simulink model "Scoped_In"  (R2025b)
settings: Solver=VariableStepAuto  StartTime=0.0  StopTime=10.0  RelTol=1e-3
settings Model: Creator=EMK7KOR  LastModifiedBy=EMK7KOR

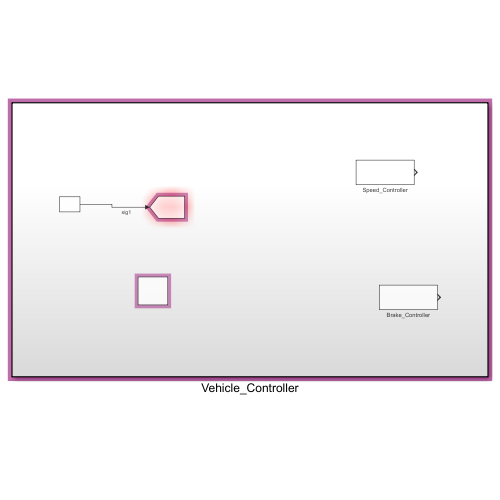
[thumbnail: Simulink's stored preview of the top-level diagram]
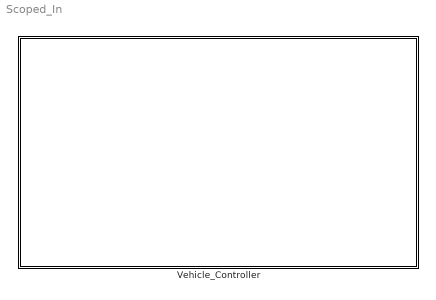
== system Scoped_In ==
  Vehicle_Controller : Subsystem

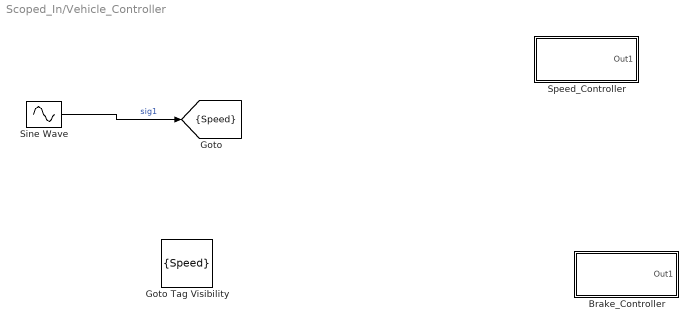
== system Scoped_In/Vehicle_Controller ==
  Brake_Controller : Subsystem
  Goto Tag Visibility : GotoTagVisibility  GotoTag=Speed
  Sine Wave : Sin  SampleTime=0
  Speed_Controller : Subsystem
  tag scope: Speed=scoped
  wires:
  Sine Wave/1 -> [Speed]  "sig1"

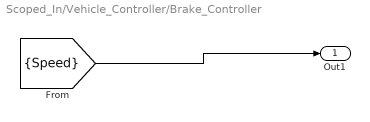
== system Scoped_In/Vehicle_Controller/Brake_Controller ==
  Out1 : Outport
  wires:
  [Speed] -> Out1/1

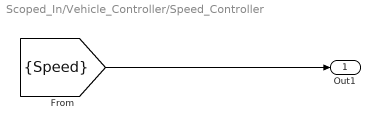
== system Scoped_In/Vehicle_Controller/Speed_Controller ==
  Out1 : Outport
  wires:
  [Speed] -> Out1/1
